simulink model "PotholeDetection3D"  (R2026b)
settings: Solver=ode23t  StopTime=13  MaxStep=0.01
undefined symbols (not defined in the file or in its folder): Sim3dSensor
libraries: dspvision x1, sim3dcameralib x1, sim3dlib x1, sim3dautolib x1
settings Model: SimulationMode=accelerator  Creator=sharm  LastModifiedBy=sharm

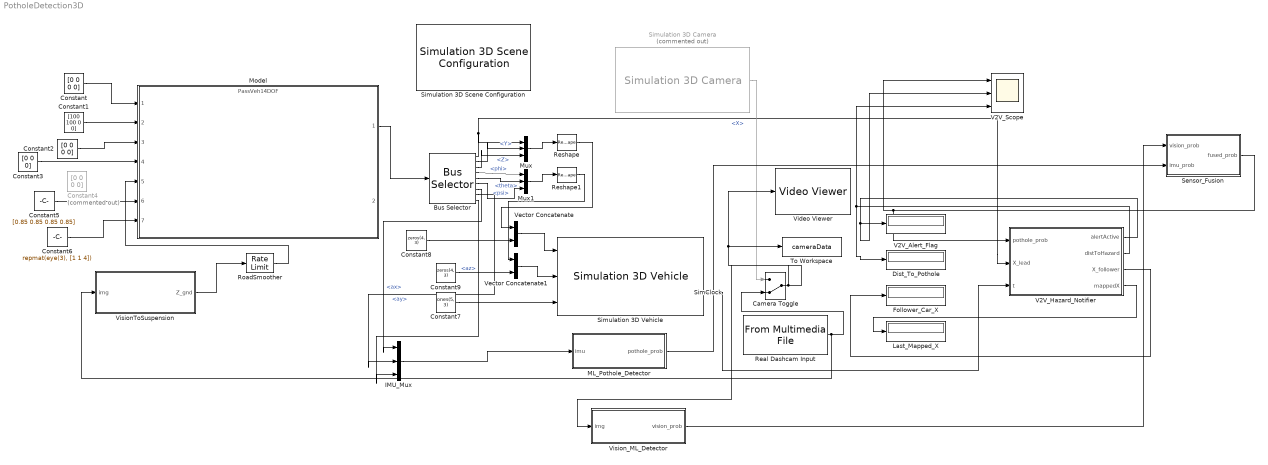
== system PotholeDetection3D ==
  Bus Selector : BusSelector  OutputSignals=InertFrm.Cg.Disp.X,InertFrm.Cg.Disp.Y,InertFrm.Cg.Disp.Z,InertFrm.Cg.Ang.phi,InertFrm.Cg.Ang.theta,InertFrm.Cg.Ang.psi,BdyFrm.Cg.Acc.ax,BdyFrm.Cg.Acc.ay,BdyFrm.Cg.Acc.az
  Camera Toggle : ManualSwitch  CurrentSetting=0
  Constant : Constant  Value=[0 0 0 0]
  Constant1 : Constant  Value=[100 100 0 0]
  Constant2 : Constant  Value=[0 0 0 0]
  Constant3 : Constant  Value=[0 0 0]
  Constant4 : Constant  Commented=on  Value=[0 0 0 0]
  Constant5 : Constant  Value=[0.85 0.85 0.85 0.85]
  Constant6 : Constant  Value=repmat(eye(3), [1 1 4])  VectorParams1D=off
  Constant7 : Constant  Value=ones(5, 3)  VectorParams1D=off
  Constant8 : Constant  Value=zeros(4, 3)  VectorParams1D=off
  Constant9 : Constant  Value=zeros(4, 3)  VectorParams1D=off
  Dist_To_Pothole : Display
  Follower_Car_X : Display
  IMU_Mux : Mux  Inputs=3
  Last_Mapped_X : Display
  ML_Pothole_Detector : MATLAB Function  TreatAsAtomicUnit=on  SystemSampleTime=1/60
  Model : ModelReference  ModelNameDialog=PassVeh14DOF.slx  SimulationMode=Normal  ModelReferenceVersion=13.6
  Mux : Mux  Inputs=3
  Mux1 : Mux  Inputs=3
  Real Dashcam Input : dspvision/From Multimedia File  inputFilename=D:\IOT PROJECT\inputs\simulink_ready_video.mp4  readRange=[1 Inf]  loop=on  numPlays=inf  outputStreams=Video only  videoDataType=single  audioDataType=int16  inheritSampleTime=on  userDefinedSampleTime=1/30  noAudioOutput=off  isIntensityVideo=off  fourcc=RGB  colorVideoFormat=One multidimensional signal  outputEOF=off  dataOrg=Column-major  audioFrameSize=1024  computeAudioFrameSize=off  outSamplingMode=Sample based
      settings: LibrarySourceBlock=visionsources/From Multimedia File
  Reshape : Reshape  OutputDimensionality=Customize  OutputDimensions=[1, 3]
  Reshape1 : Reshape  OutputDimensionality=Customize  OutputDimensions=[1, 3]
  RoadSmoother : RateLimiter  RisingSlewLimit=6.0  FallingSlewLimit=-6.0  SampleTimeMode=inherited
  Sensor_Fusion : MATLAB Function  TreatAsAtomicUnit=on  SystemSampleTime=1/60
  SimClock : Clock
  Simulation 3D Camera : sim3dcameralib/Simulation 3D Camera  Priority=1  Commented=on  sensorTag=Sim3dSensor�  sensorId=1  sensorName=Sim3dSensor�  vehTagList={'Custom ...';'Scene Origin';'SimulinkVehicle2'}  vehTag=SimulinkVehicle2  CoordinateSystem=ISO8855  mountLoc=Front bumper  offsetFlag=off  tmountOffset=[0, 0, 0]  extTmount=off  rmountOffset=[0, 0, 0]  extRmount=off  FocalLength=[1109, 1109]  OpticalCenter=[640, 360]  ImageSize=[480 640]  RadialDistortion=[0, 0]  TangentialDistortion=[0, 0]  SensorSkew=0  VisualizeFieldOfView=on  FieldOfViewRange=61  DepthOutportEnabled=off  SemanticOutportEnabled=off  TransformOutportEnabled=off  SampleTime=-1  mountPoint=[2.424 0 0.5]  mountOrientation=[0 0 0]  aMode=3  ID=1
      settings: LibrarySourceBlock=drivingsim3d/Simulation 3D Camera
  Simulation 3D Scene Configuration : sim3dlib/Simulation 3D Scene Configuration  Priority=0  EnableWindow=on  ViewerType=Default Viewer  ProjectFormat=Default Scenes  SceneDesc=Straight road  ProjectName=C:\Program Files\MATLAB\R2026b\toolbox\shared\sim3d_projects\automotive_project_windows\UE\WindowsNoEditor\VehicleSimulation.exe  ScenePath=/Game/Maps/HwStrght  EnableOpenDRIVE=off  vehTagList={'Custom';'Scene Origin';'SimulinkVehicle2'}  vehTag=SimulinkVehicle2  AttachedCameraRelativeTranslation=[0 0 0]  FreeCameraDefaultInitialTranslation=[-6, 0, 2]  AttachedCameraRelativeRotation=[0, -15, 0]  FreeCameraDefaultInitialRotation=[0, -15, 0]  ViewpointName=Custom  FreeCameraInitialTranslation=[0, 0, 0]  FreeCameraInitialRotation=[0, 0, 0]  OpVisEn=off  Ts=1/30  EnableRemoteAccess=off  SimulationMode=CoSimulation  SimulateUsing=Interpreted execution  EnableAnimationRecording=off  OverrideDefaultRecording=off  AnimationRecordingFileName=sim3dAnimation.mat  AnimationRecordingInterval=[0 inf]  EnableWeather=off  SunAzimuth=90  SunAltitude=40.0  EnableGeospatialSun=off  Latitude=0  Longitude=0  Date=2023-01-01  Time=10:30:00  GeoTimeZone=-5.0  SunDaylightSaving=off  wind=1  clouds=10  EnableVolumetricClouds=off  CloudCoverage=0  CloudAltitude=6  fog=0  rain=0  RaindropsEffect=off  SnowDensity=0  EnableGeospatial=off  TilesetSource=Earth terrain  UseTrueOrigin=off  OriginHeight=200  OriginLatitude=40.744652  OriginLongitude=-73.988864  MapStyle=Aerial  AdditionalAssetIDs=[]  UseAdvancedSunSky=off  SolarTime=11  TimeZone=-5  Day=21  Month=9  Year=2022  UseDaylightSavingTime=on  DSTStartDay=10  DSTStartMonth=3  DSTEndDay=3  DSTEndMonth=11  DSTSwitchHour=2  sensorTag=MainCamera1  sensorId=1  sensorName=MainCamera1  mountLoc=Origin  offsetFlag=off  tmountOffset=[0, 0, 0]  rmountOffset=[0, 0, 0]  HorizontalResolution=1280  VerticalResolution=720  HorizontalFOV=60  mountPoint=[0 0 0]  mountOrientation=[0 0 0]  aMode=3  ID=1  GeoTrigger=Inactive  ViewNameList={'Custom'}  ViewTranslationList={'[0 0 0]'}  ViewRotationList={'[0 0 0]'}
      settings: LibrarySourceBlock=drivingsim3d/Simulation 3D Scene Configuration
  Simulation 3D Vehicle : sim3dautolib/Simulation 3D Vehicle  Priority=-1  PassVehMesh=Sedan  MeshPath=/MathWorksAutomotiveContent/Vehicles/Muscle/Meshes/SK_MuscleCar.SK_MuscleCar  VehColor=Red  ActorName=SimulinkVehicle2  VehLightsControl=off  HeadlightColor=[ 1, 1, 1 ]  HighBeamIntensity=100000  LowBeamIntensity=60000  HighBeamConeAngle=1.22  LowBeamConeAngle=1.22  LeftHeadlightOrientation=[ 0, 0 ]  RightHeadlightOrientation=[ 0, 0 ]  BrakelightIntensity=500  ReverselightIntensity=500  SignallightIntensity=500  SignallightPeriod=1  SignalPulseWidth=50  Translation=zeros( 5, 3 )  Rotation=zeros( 5, 3 )  Scale=ones( 5, 3 )  SampleTime=-1  ActorType=SimulinkVehicle  ID=2  aMode=2  ActorTag=SimulinkVehicle2
      settings: LibrarySourceBlock=vehdynlibsim3d/Simulation 3D Vehicle
  To Workspace : ToWorkspace  VariableName=cameraData  SaveFormat=Timeseries  SampleTime=-1
  V2V_Alert_Flag : Display
  V2V_Hazard_Notifier : MATLAB Function  TreatAsAtomicUnit=on  SystemSampleTime=1/60
  V2V_Scope : Scope  NumInputPorts=3
      settings: ActiveDisplayYMinimum=-0.11490768607130428  ActiveDisplayYMaximum=1.1234438622612319
  Vector Concatenate : Concatenate  Mode=Multidimensional array
  Vector Concatenate1 : Concatenate  Mode=Multidimensional array
  Video Viewer : VideoViewer  FigPos=[956 504 418 304]
  VisionToSuspension : MATLAB Function  TreatAsAtomicUnit=on
  Vision_ML_Detector : MATLAB Function  TreatAsAtomicUnit=on  SystemSampleTime=1/60
  wires:
  Constant/1 -> Model/1
  Constant1/1 -> Model/2
  Constant2/1 -> Model/3
  Constant3/1 -> Model/4
  Constant5/1 -> Model/6
  Constant6/1 -> Model/7
  Model/1 -> Bus Selector/1
  Constant7/1 -> Simulation 3D Vehicle/3
  Bus Selector/1 -> Mux/1, V2V_Hazard_Notifier/2(X_lead)  "<X>"
  Bus Selector/2 -> Mux/2  "<Y>"
  Bus Selector/3 -> Mux/3  "<Z>"
  Bus Selector/4 -> Mux1/1  "<phi>"
  Bus Selector/5 -> Mux1/2  "<theta>"
  Bus Selector/6 -> Mux1/3  "<psi>"
  Mux/1 -> Reshape/1
  Mux1/1 -> Reshape1/1
  Reshape/1 -> Vector Concatenate/1
  Constant8/1 -> Vector Concatenate/2
  Vector Concatenate/1 -> Simulation 3D Vehicle/1
  Reshape1/1 -> Vector Concatenate1/1
  Constant9/1 -> Vector Concatenate1/2
  Vector Concatenate1/1 -> Simulation 3D Vehicle/2
  Simulation 3D Camera/1 -> Camera Toggle/1
  Real Dashcam Input/1 -> Camera Toggle/2, VisionToSuspension/1(img)
  Camera Toggle/1 -> Video Viewer/1, To Workspace/1, Vision_ML_Detector/1(img)
  VisionToSuspension/1(Z_gnd) -> RoadSmoother/1
  RoadSmoother/1 -> Model/5
  Bus Selector/7 -> IMU_Mux/1  "<ax>"
  Bus Selector/8 -> IMU_Mux/2  "<ay>"
  Bus Selector/9 -> IMU_Mux/3  "<az>"
  IMU_Mux/1 -> ML_Pothole_Detector/1(imu)
  ML_Pothole_Detector/1(pothole_prob) -> Sensor_Fusion/2(imu_prob)
  SimClock/1 -> V2V_Hazard_Notifier/3(t)
  V2V_Hazard_Notifier/1(alertActive) -> V2V_Scope/2, V2V_Alert_Flag/1
  V2V_Hazard_Notifier/2(distToHazard) -> Dist_To_Pothole/1, V2V_Scope/3
  V2V_Hazard_Notifier/3(X_follower) -> Follower_Car_X/1
  V2V_Hazard_Notifier/4(mappedX) -> Last_Mapped_X/1
  Vision_ML_Detector/1(vision_prob) -> Sensor_Fusion/1(vision_prob)
  Sensor_Fusion/1(fused_prob) -> V2V_Scope/1, V2V_Hazard_Notifier/1(pothole_prob)

== matlab function PotholeDetection3D/ML_Pothole_Detector ==
  data: imu input; pothole_prob output
function pothole_prob = ML_Pothole_Detector(imu)
coder.extrinsic('run_pothole_lstm');
persistent win
if isempty(win)
    win = zeros(30, 3);
end

% Shift 30-sample sliding window [ax, ay, az]
win(1:end-1, :) = win(2:end, :);
win(end, :) = imu(:)';

% Mean-center window to match Colab preprocessing
win_norm = win - mean(win, 1);

% Pre-allocate output type/size for Simulink, then call LSTM
pothole_prob = 0.0;
pothole_prob = run_pothole_lstm(win_norm);
end

== matlab function PotholeDetection3D/VisionToSuspension ==
  data: img input; Z_gnd output
function Z_gnd = VisionToSuspension(img)
roi_L = double(img(360:4:470, 50:4:260, :));
roi_R = double(img(360:4:470, 380:4:590, :));
gray_L = roi_L(:,:,1)*0.299 + roi_L(:,:,2)*0.587 + roi_L(:,:,3)*0.114;
gray_R = roi_R(:,:,1)*0.299 + roi_R(:,:,2)*0.587 + roi_R(:,:,3)*0.114;
mL = mean(gray_L(:)); mR = mean(gray_R(:));
dL = sum(gray_L(:) > mL*1.45 | gray_L(:) < mL*0.50) / numel(gray_L);
dR = sum(gray_R(:) > mR*1.45 | gray_R(:) < mR*0.50) / numel(gray_R);
z_FL = -0.12 * min(1.0, max(0.0, (dL - 0.03) / 0.20));
z_FR = -0.12 * min(1.0, max(0.0, (dR - 0.03) / 0.20));
persistent z_hist
if isempty(z_hist), z_hist = zeros(12, 2); end
z_RL = z_hist(1,1); z_RR = z_hist(1,2);
z_hist(1:end-1,:) = z_hist(2:end,:);
z_hist(end,:) = [z_FL, z_FR];
Z_gnd = [z_FL, z_FR, z_RL, z_RR];
end

== matlab function PotholeDetection3D/V2V_Hazard_Notifier ==
  data: pothole_prob input; alertActive output; X_lead input; t input; distToHazard output; X_follower output; mappedX output
function [alertActive, distToHazard, X_follower, mappedX] = V2V_Hazard_Notifier(pothole_prob, X_lead, t)
persistent hazardList count followerX followerV lastT
if isempty(hazardList)
    hazardList = zeros(1, 50);
    count = 0;
    followerX = -35.0; % Start 35 m behind lead car
    followerV = 14.0;
    lastT = 0.0;
end
dt = max(0.0, t - lastT);
lastT = t;

% Sync lead car road position with dashcam speed (14 m/s ~ 50 km/h)
leadX = max(X_lead, 14.0 * t);

% 1. Map pothole when fused probability > 0.55 (min 20 m spacing)
if pothole_prob > 0.65
    if count == 0 || abs(leadX - hazardList(count)) > 20.0
        if count < 50
            count = count + 1;
            hazardList(count) = leadX;
        end
    end
end

% 2. Find nearest upcoming mapped pothole ahead of follower car
alertActive = 0;
distToHazard = 999.0;
mappedX = 0.0;
if count > 0
    mappedX = hazardList(count);
end
for i = 1:count
    d = hazardList(i) - followerX;
    if d > 0 && d < distToHazard
        distToHazard = d;
    end
end

% 3. V2V Alert & Braking within 18 m
if distToHazard <= 10.0
    alertActive = 1;
    followerV = max(8.0, followerV - 4.0 * dt);
else
    followerV = min(14.0, followerV + 3.0 * dt);
end
followerX = min(followerX + followerV * dt, leadX - 25.0);
X_follower = followerX;
end

== matlab function PotholeDetection3D/Vision_ML_Detector ==
  data: img input; vision_prob output
function vision_prob = Vision_ML_Detector(img)
coder.extrinsic('run_pothole_yolo');
vision_prob = 0.0;
vision_prob = run_pothole_yolo(img);
end

== matlab function PotholeDetection3D/Sensor_Fusion ==
  data: vision_prob input; fused_prob output; imu_prob input
function fused_prob = Sensor_Fusion(vision_prob, imu_prob)
% Camera sees pothole ~0.5-1.5s BEFORE the tires hit it.
% Hold peak vision confidence briefly so it aligns with the IMU jolt.
persistent vis_hold
if isempty(vis_hold), vis_hold = 0.0; end
vis_hold = max(vision_prob, vis_hold * 0.96); % ~1.5s decay at 60 Hz

% Late-fusion confidence score
fused_prob = min(1.0, 0.45 * vis_hold + 0.55 * imu_prob);
end
